simulink model "BLDC_MOTOR_ASW"  (R2023b)
settings: Solver=FixedStepDiscrete  StartTime=0.0  StopTime=10.0  FixedStep=1e-4  RelTol=1e-3
undefined symbols (not defined in the file): D1, P
settings Model: DataDictionary=Arch.sldd  Creator=84339  LastModifiedBy=84339
settings OptimizationCC: DefaultParameterBehavior=Inlined  EnhancedBackFolding=on  PassReuseOutputArgsAs=Individual arguments  ZeroExternalMemoryAtStartup=off  ZeroInternalMemoryAtStartup=off  OptimizeBlockOrder=speed  DifferentSizesBufferReuse=on  OptimizationCustomize=off  EfficientTunableParamExpr=on
settings DebuggingCC: ParameterTunabilityLossMsg=error
settings SFSimCC: MATLABDynamicMemAlloc=off
settings RTWCC: Description=Embedded Coder  SystemTargetFile=ert.tlc  EmbeddedCoderDictionary=Arch.sldd  GenCodeOnly=on  TemplateMakefile=ert_default_tmf
settings CodeAppCC: ForceParamTrailComments=on  IgnoreCustomStorageClasses=off  OperatorAnnotations=on  SimulinkDataObjDesc=on  SFDataObjDesc=on  InsertBlockDesc=on
settings ERTTargetCC: TargetLangStandard=C99 (ISO)  GenerateSampleERTMain=on  InlinedParameterPlacement=NonHierarchical  ERTCustomFileTemplate=example_file_process.tlc

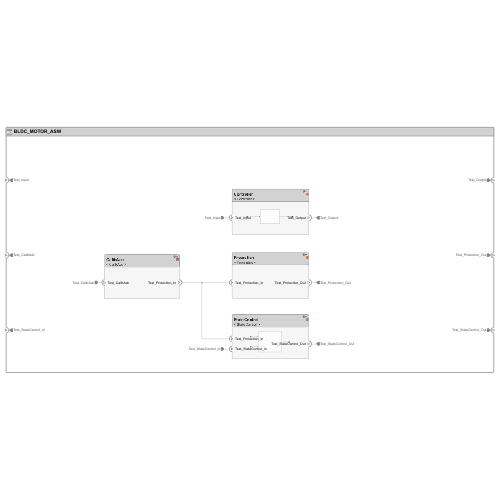
[thumbnail: Simulink's stored preview of the top-level diagram]
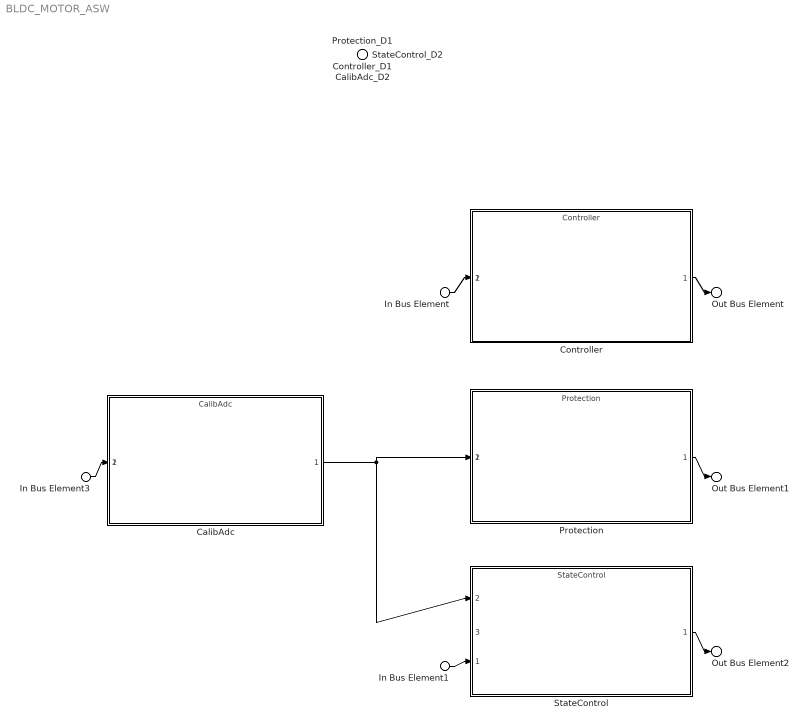
== system BLDC_MOTOR_ASW ==
  In Bus Element : Inport  PortName=Test_Input
  In Bus Element3 : Inport  Port=2  PortName=Test_CalibAdc
  In Bus Element1 : Inport  Port=3  PortName=Test_StateControl_In
  Controller_D1 : Inport  Port=4  OutputFunctionCall=on
  Protection_D1 : Inport  Port=5  OutputFunctionCall=on
  CalibAdc_D2 : Inport  Port=6  OutputFunctionCall=on
  StateControl_D2 : Inport  Port=7  OutputFunctionCall=on
  CalibAdc : ModelReference  ModelNameDialog=CalibAdc.slx  SimulationMode=Normal  ScheduleRates=on  CachedPortDiscreteRates=[0.0001]  ModelEventPortInfo=P:D1[0.0001][0][0]  ModelReferenceVersion=1.51
      settings: PortSchema="{\"entries\":[{\"content\":{\"headerSize\":38,\"margin\":15,\"minimumSpacing\":25,\"sides\":[{\"content\":{\"connectorIds\":[\"In1\"]},\"type\":\"ConnectorPlacement.EquallySpacedRectSide\",\"uuid\":\"af89fbb1-38b7-40cd-b67d-0ae5a9769455\"},{\"content\":{\"connectorIds\":[\"Out1\"],\"side\":\"RIGHT\"},\"type\":\"ConnectorPlacement.EquallySpacedRectSide\",\"uuid\":\"95c6f8f6-ab64-41cf-8b6e-03d5f7ff20c2\"},{\"content\":{\"side\":\"TOP\"},\"type\":\"ConnectorPlacement.EquallySpacedRectSide\",\"uuid\":\"3088db2c-f0cc-43dd-896c-d3fe2b9a560c\"},{\"content\":{\"connectorIds\":[\"In2\"],\"side\":\"HIDDEN\"},\"type\":\"ConnectorPlacement.EquallySpacedRectSide\",\"uuid\":\"9c054a74-60ce-4428-b28c-f5f1f1b57afd\"}]},\"type\":\"ConnectorPlacement.EquallySpacedConnector\",\"uuid\":\"821c2a66-3465-4843-859e-4a5701700f54\"}],\"packageUris\":[\"http://schema.mathworks.com/mf0/Connector/R2020b\"],\"version\":\"1.0\"}"
  Controller : ModelReference  ModelNameDialog=Controller.slx  SimulationMode=Normal  ScheduleRates=on  CachedPortDiscreteRates=[0.0001]  ModelEventPortInfo=P:D1[0.0001][0][0]  ModelReferenceVersion=1.186
      settings: PortSchema="{\"entries\":[{\"content\":{\"headerSize\":38,\"margin\":15,\"minimumSpacing\":25,\"sides\":[{\"content\":{\"connectorIds\":[\"In1\"]},\"type\":\"ConnectorPlacement.EquallySpacedRectSide\",\"uuid\":\"9c5e37b8-ebc1-4039-8efe-be9823ad02d8\"},{\"content\":{\"connectorIds\":[\"Out1\"],\"side\":\"RIGHT\"},\"type\":\"ConnectorPlacement.EquallySpacedRectSide\",\"uuid\":\"af13a687-424c-4511-9bac-72719f846905\"},{\"content\":{\"side\":\"TOP\"},\"type\":\"ConnectorPlacement.EquallySpacedRectSide\",\"uuid\":\"c0e5a812-d245-4d86-a4cd-e2bd34812cf3\"},{\"content\":{\"connectorIds\":[\"In2\"],\"side\":\"HIDDEN\"},\"type\":\"ConnectorPlacement.EquallySpacedRectSide\",\"uuid\":\"4c8d37c3-ad5b-497f-a802-5d32e1cb9856\"}]},\"type\":\"ConnectorPlacement.EquallySpacedConnector\",\"uuid\":\"026f73d4-5d51-4722-964e-695994d5c3be\"}],\"packageUris\":[\"http://schema.mathworks.com/mf0/Connector/R2020b\"],\"version\":\"1.0\"}"
  Protection : ModelReference  ModelNameDialog=Protection.slx  SimulationMode=Normal  ScheduleRates=on  CachedPortDiscreteRates=[0.0001]  ModelEventPortInfo=P:D1[0.0001][0][0]  ModelReferenceVersion=1.53
      settings: PortSchema="{\"entries\":[{\"content\":{\"headerSize\":38,\"margin\":15,\"minimumSpacing\":25,\"sides\":[{\"content\":{\"connectorIds\":[\"In1\"]},\"type\":\"ConnectorPlacement.EquallySpacedRectSide\",\"uuid\":\"315ad4a0-b464-4891-ad59-f68b1663d8e6\"},{\"content\":{\"connectorIds\":[\"Out1\"],\"side\":\"RIGHT\"},\"type\":\"ConnectorPlacement.EquallySpacedRectSide\",\"uuid\":\"310e912b-1e65-4313-a75b-4f71cb84b04e\"},{\"content\":{\"side\":\"TOP\"},\"type\":\"ConnectorPlacement.EquallySpacedRectSide\",\"uuid\":\"5af11a9a-b24b-4ecf-b54c-f88f43e95791\"},{\"content\":{\"connectorIds\":[\"In2\"],\"side\":\"HIDDEN\"},\"type\":\"ConnectorPlacement.EquallySpacedRectSide\",\"uuid\":\"529ffeab-9d81-4c80-b1cb-70eb0bc0c062\"}]},\"type\":\"ConnectorPlacement.EquallySpacedConnector\",\"uuid\":\"8b6093a8-c5b1-4e91-bd44-ed7a4f1897e3\"}],\"packageUris\":[\"http://schema.mathworks.com/mf0/Connector/R2020b\"],\"version\":\"1.0\"}"
  StateControl : ModelReference  ModelNameDialog=StateControl.slx  SimulationMode=Normal  ScheduleRates=on  CachedPortDiscreteRates=[0.0001]  ModelEventPortInfo=P:D1[0.0001][0][0]  ModelReferenceVersion=1.40
      settings: PortSchema="{\"entries\":[{\"content\":{\"headerSize\":38,\"margin\":15,\"minimumSpacing\":25,\"sides\":[{\"content\":{\"connectorIds\":[\"In2\",\"In1\"]},\"type\":\"ConnectorPlacement.EquallySpacedRectSide\",\"uuid\":\"8be39887-5270-4598-a925-15c2b5cb83bd\"},{\"content\":{\"connectorIds\":[\"Out1\"],\"side\":\"RIGHT\"},\"type\":\"ConnectorPlacement.EquallySpacedRectSide\",\"uuid\":\"8874901c-8238-4768-b8db-855ef83702a2\"},{\"content\":{\"side\":\"TOP\"},\"type\":\"ConnectorPlacement.EquallySpacedRectSide\",\"uuid\":\"7d402af2-4a94-41f1-b9cc-6291402e3c39\"},{\"content\":{\"connectorIds\":[\"In3\"],\"side\":\"HIDDEN\"},\"type\":\"ConnectorPlacement.EquallySpacedRectSide\",\"uuid\":\"be29f021-980f-4877-aea4-75f3ff3756ec\"}]},\"type\":\"ConnectorPlacement.EquallySpacedConnector\",\"uuid\":\"1757bdec-f6b1-47dc-81d2-8f4b29413c9a\"}],\"packageUris\":[\"http://schema.mathworks.com/mf0/Connector/R2020b\"],\"version\":\"1.0\"}"
  Out Bus Element : Outport  PortName=Test_Output
  Out Bus Element1 : Outport  Port=2  PortName=Test_Protection_Out
  Out Bus Element2 : Outport  Port=3  PortName=Test_StateControl_Out
  wires:
  In Bus Element/1 -> Controller/1
  Controller/1 -> Out Bus Element/1
  Protection/1 -> Out Bus Element1/1
  In Bus Element1/1 -> StateControl/1
  StateControl/1 -> Out Bus Element2/1
  In Bus Element3/1 -> CalibAdc/1
  CalibAdc/1 -> StateControl/2, Protection/1
